simulink model "W06_7_front_vrx"  (R2024b)
settings: Solver=ode4  StartTime=0.0  StopTime=T_run  FixedStep=Ts_ctrl  RelTol=1e-3
InitFcn:
  | if ~exist('W06_model_init','file'), addpath(fileparts(get_param('W06_7_front_vrx','FileName'))); end, W06_model_init('W06_7_front_vrx')
StopFcn:
  | W06_model_done('W06_7_front_vrx')
values from neighbouring files (symbols this model uses):
  alloc_prm = [half_beam; l_bow; F_max; F_bow_max]    [W06_setup.m]
  animate = 0    [W06_bow_demo.m]    (also in W06_psi_sweep.m; W06_setup.m = 1)
  bow_on = BOW(i)    [W06_bow_demo.m]    (also in W06_setup.m = 1)
  F_bow_max = 250    [W06_setup.m]
  F_max = 500    [W06_setup.m]
  F_plugin_max = 2353.53383667818    (= 2353.53383668)    [W06_setup.m]
  half_beam = 1.027135    [W06_setup.m]
  k_prop = 1000 * 0.004422 * 0.2^4    (= 0.0070752)    [W06_setup.m]
  Kb = Ki_u / Kp_u    (= 0.333333333333)    [W06_setup.m]
  Kd_psi = 200    [W06_setup.m]
  Ki_u = 100    [W06_setup.m]
  Ki_v = 100    [W06_setup.m]
  Kp_psi = 400    [W06_setup.m]
  Kp_u = 300    [W06_setup.m]
  Kp_v = 300    [W06_setup.m]
  Kp_x = 0.4    [W06_setup.m]
  Kp_y = 0.4    [W06_setup.m]
  l_bow = 0.75    [W06_setup.m]
  origin_east = -532    [W06_setup.m]
  origin_north = 200    [W06_setup.m]
  stop_hold = 15    [W06_setup.m]
  task_q = [ hold_north;  hold_east;  deg2rad(hold_deg) ... (first row only)    [W06_setup.m]
  Ts_ctrl = 0.05    [W06_setup.m]
  u_max = 1.5    [W06_setup.m]
  v_max = 0.6    [W06_setup.m]
libraries: ros2lib x7, slpidlib x2
settings Model: Creator=admin  LastModifiedBy=admin

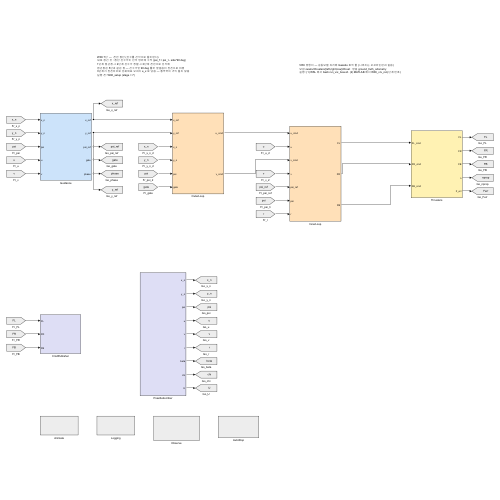
[thumbnail: Simulink's stored preview of the top-level diagram]
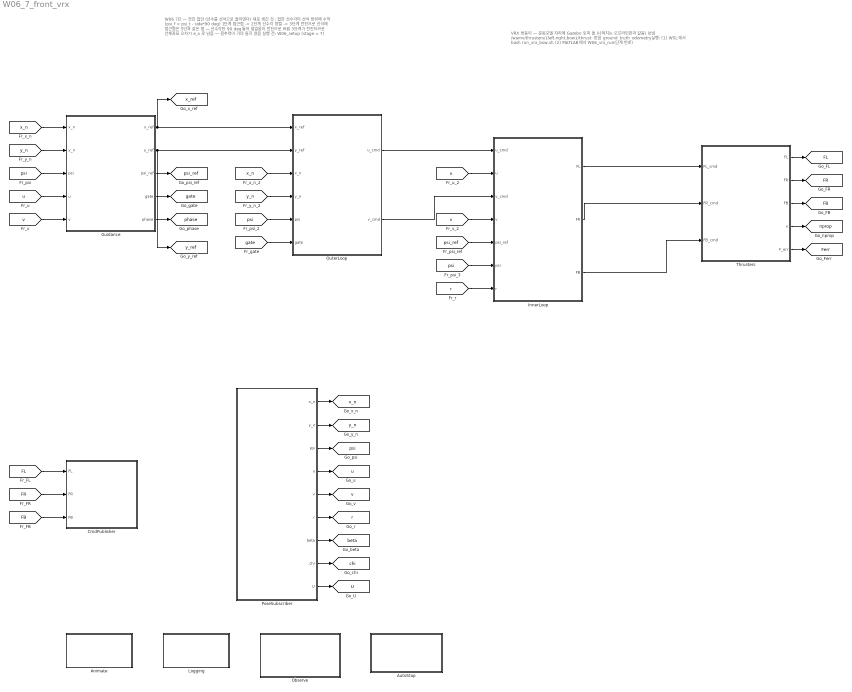
== system W06_7_front_vrx ==
  note: VRX 쌍둥이 — 운동모델 자리에 Gazebo 토픽 둘 (나머지는 오프라인판과 같음)
      | 보냄 /wamv/thrusters/{left,right,bow}/thrust · 받음 ground_truth_odometry
      | 실행: (1) WSL 에서 bash run_vrx_bow.sh  (2) MATLAB 에서 W06_vrx_run(단계 번호)
  note: W06 7단  —  전진 접안 (선수를 선석으로 들이댄다)
      | 새로 생긴 것 : 접안 선수각이 선석 방위에 수직 (psi_f = psi_t - side*90 deg)
      | 1단계 접근점 -> 2단계 선수각 정렬 -> 3단계 전진으로 선석에
      | 접근점은 5단과 같은 점 — 선수각만 90 deg 틀어 옆걸음이 전진으로 바뀜
      | 3단계가 전진이므로 선체좌표 오차가 e_x 로 남음 — 횡추력이 거의 들지 않음
      | 실행 전: W06_setup (stage = 7)
  Animate : Subsystem
  AutoStop : Subsystem
  CmdPublisher : Subsystem
  Guidance : Subsystem
  InnerLoop : Subsystem
  Logging : Subsystem
  Observe : Subsystem
  OuterLoop : Subsystem
  PoseSubscriber : Subsystem
  Thrusters : Subsystem
  tag scope: FB=global, FL=global, FR=global, Ferr=global, U=global, beta=global, chi=global, gate=global, nprop=global, phase=global, psi=global, psi_ref=global, r=global, u=global, v=global, x_n=global, x_ref=global, y_n=global, y_ref=global
  wires:
  InnerLoop/3(FB) -> Thrusters/3(FB_cmd)
  InnerLoop/2(FR) -> Thrusters/2(FR_cmd)
  InnerLoop/1(FL) -> Thrusters/1(FL_cmd)
  OuterLoop/2(v_cmd) -> InnerLoop/3(v_cmd)
  OuterLoop/1(u_cmd) -> InnerLoop/1(u_cmd)
  Guidance/1(x_ref) -> OuterLoop/1(x_ref), [x_ref]
  Guidance/2(y_ref) -> OuterLoop/2(y_ref), [y_ref]
  Thrusters/1(FL) -> [FL]
  Thrusters/2(FR) -> [FR]
  Thrusters/4(n) -> [nprop]
  PoseSubscriber/3(psi) -> [psi]
  Guidance/3(psi_ref) -> [psi_ref]
  PoseSubscriber/6(r) -> [r]
  PoseSubscriber/4(u) -> [u]
  PoseSubscriber/5(v) -> [v]
  PoseSubscriber/1(x_n) -> [x_n]
  PoseSubscriber/2(y_n) -> [y_n]
  [FB] -> CmdPublisher/3(FB)
  [FL] -> CmdPublisher/1(FL)
  [FR] -> CmdPublisher/2(FR)
  [psi_ref] -> InnerLoop/5(psi_ref)
  [r] -> InnerLoop/7(r)
  [u] -> InnerLoop/2(u)
  [v] -> Guidance/5(v)
  [v] -> InnerLoop/4(v)
  [x_n] -> Guidance/1(x_n)
  [y_n] -> Guidance/2(y_n)
  Thrusters/3(FB) -> [FB]
  Thrusters/5(F_err) -> [Ferr]
  PoseSubscriber/9(U) -> [U]
  PoseSubscriber/7(beta) -> [beta]
  PoseSubscriber/8(chi) -> [chi]
  Guidance/4(gate) -> [gate]
  Guidance/5(phase) -> [phase]
  [gate] -> OuterLoop/6(gate)
  [psi] -> Guidance/3(psi)
  [psi] -> InnerLoop/6(psi)
  [u] -> Guidance/4(u)
  [x_n] -> OuterLoop/3(x_n)
  [y_n] -> OuterLoop/4(y_n)
  [psi] -> OuterLoop/5(psi)

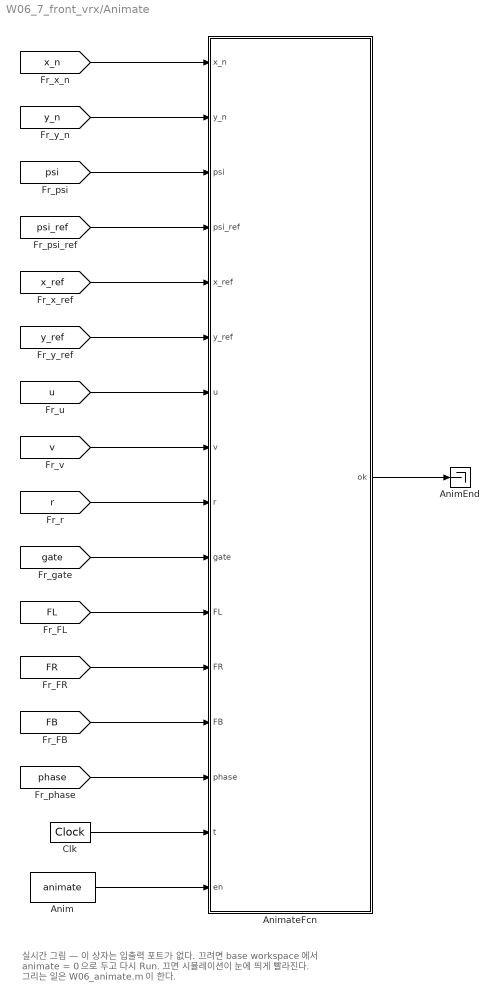
== system W06_7_front_vrx/Animate ==
  note: 실시간 그림 — 이 상자는 입출력 포트가 없다.
      | 끄려면 base workspace 에서  animate = 0  으로 두고 다시 Run.
      | 끄면 시뮬레이션이 눈에 띄게 빨라진다.
      | 그리는 일은 W06_animate.m 이 한다.
  Anim : Constant  Value=animate
  AnimEnd : Terminator
  AnimateFcn : MATLAB Function  TreatAsAtomicUnit=on
  Clk : DigitalClock  SampleTime=Ts_ctrl
  wires:
  [x_n] -> AnimateFcn/1(x_n)
  [y_n] -> AnimateFcn/2(y_n)
  [psi] -> AnimateFcn/3(psi)
  [psi_ref] -> AnimateFcn/4(psi_ref)
  [x_ref] -> AnimateFcn/5(x_ref)
  [y_ref] -> AnimateFcn/6(y_ref)
  [u] -> AnimateFcn/7(u)
  [v] -> AnimateFcn/8(v)
  [r] -> AnimateFcn/9(r)
  [gate] -> AnimateFcn/10(gate)
  [FL] -> AnimateFcn/11(FL)
  [FR] -> AnimateFcn/12(FR)
  [FB] -> AnimateFcn/13(FB)
  [phase] -> AnimateFcn/14(phase)
  Clk/1 -> AnimateFcn/15(t)
  Anim/1 -> AnimateFcn/16(en)
  AnimateFcn/1(ok) -> AnimEnd/1

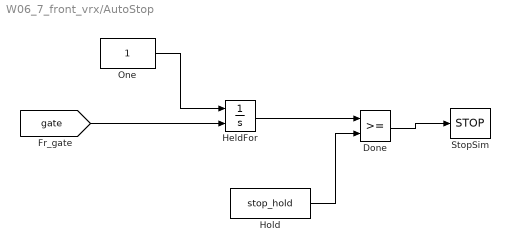
== system W06_7_front_vrx/AutoStop ==
  Done : RelationalOperator  OutDataTypeStr=boolean  RndMeth=Simplest  InputSameDT=off
  HeldFor : Integrator  ExternalReset=level
  Hold : Constant  Value=stop_hold
  One : Constant
  StopSim : Stop
  wires:
  One/1 -> HeldFor/1
  [gate] -> HeldFor/2
  HeldFor/1 -> Done/1
  Hold/1 -> Done/2
  Done/1 -> StopSim/1

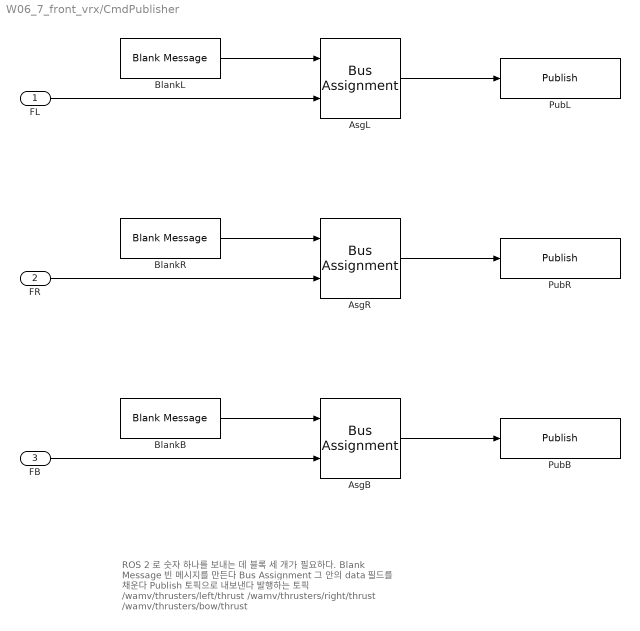
== system W06_7_front_vrx/CmdPublisher ==
  note: ROS 2 로 숫자 하나를 보내는 데 블록 세 개가 필요하다.
      |   Blank Message   빈 메시지를 만든다
      |   Bus Assignment  그 안의 data 필드를 채운다
      |   Publish         토픽으로 내보낸다
      |
      | 발행하는 토픽
      | /wamv/thrusters/left/thrust
      | /wamv/thrusters/right/thrust
      | /wamv/thrusters/bow/thrust
  FL : Inport
  FR : Inport  Port=2
  FB : Inport  Port=3
  AsgB : BusAssignment  AssignedSignals=data
  AsgL : BusAssignment  AssignedSignals=data
  AsgR : BusAssignment  AssignedSignals=data
  BlankB : ros2lib/Blank Message  messageClass=Message  entityType=std_msgs/Float64  messageType=std_msgs/Float64  SampleTime=Ts_ctrl
  BlankL : ros2lib/Blank Message  messageClass=Message  entityType=std_msgs/Float64  messageType=std_msgs/Float64  SampleTime=Ts_ctrl
  BlankR : ros2lib/Blank Message  messageClass=Message  entityType=std_msgs/Float64  messageType=std_msgs/Float64  SampleTime=Ts_ctrl
  PubB : ros2lib/Publish  topicSource=Specify your own  topic=/wamv/thrusters/bow/thrust  messageType=std_msgs/Float64  QOSHistory=Keep last  QOSDepth=1  QOSReliability=Reliable  QOSDurability=Volatile  QOSDeadline=Inf  QOSLifespan=Inf  QOSLiveliness=Automatic  QOSLeaseDuration=Inf  QOSAvoidROSNamespaceConventions=off
  PubL : ros2lib/Publish  topicSource=Specify your own  topic=/wamv/thrusters/left/thrust  messageType=std_msgs/Float64  QOSHistory=Keep last  QOSDepth=1  QOSReliability=Reliable  QOSDurability=Volatile  QOSDeadline=Inf  QOSLifespan=Inf  QOSLiveliness=Automatic  QOSLeaseDuration=Inf  QOSAvoidROSNamespaceConventions=off
  PubR : ros2lib/Publish  topicSource=Specify your own  topic=/wamv/thrusters/right/thrust  messageType=std_msgs/Float64  QOSHistory=Keep last  QOSDepth=1  QOSReliability=Reliable  QOSDurability=Volatile  QOSDeadline=Inf  QOSLifespan=Inf  QOSLiveliness=Automatic  QOSLeaseDuration=Inf  QOSAvoidROSNamespaceConventions=off
  wires:
  BlankL/1 -> AsgL/1
  AsgL/1 -> PubL/1
  FL/1 -> AsgL/2
  BlankR/1 -> AsgR/1
  AsgR/1 -> PubR/1
  FR/1 -> AsgR/2
  BlankB/1 -> AsgB/1
  AsgB/1 -> PubB/1
  FB/1 -> AsgB/2

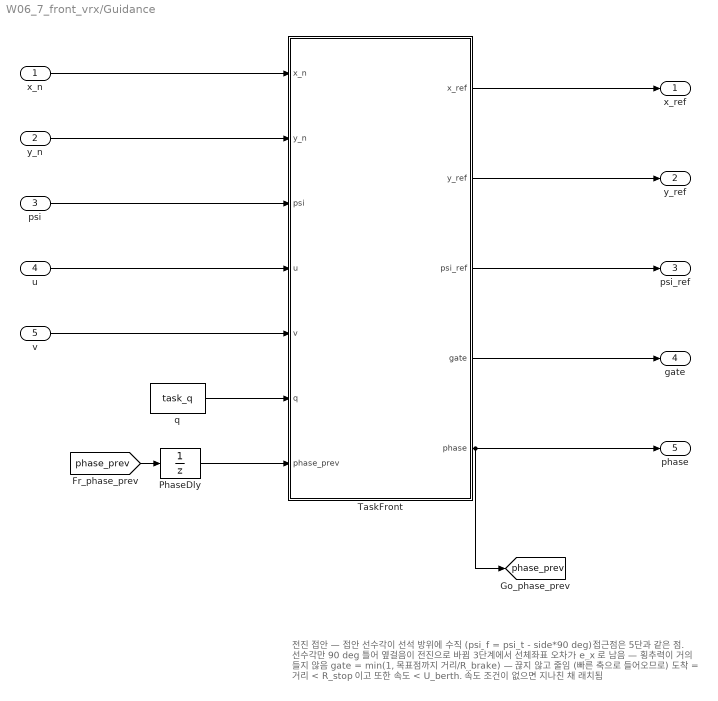
== system W06_7_front_vrx/Guidance ==
  note: 전진 접안 — 접안 선수각이 선석 방위에 수직 (psi_f = psi_t - side*90 deg)
      | 접근점은 5단과 같은 점. 선수각만 90 deg 틀어 옆걸음이 전진으로 바뀜
      | 3단계에서 선체좌표 오차가 e_x 로 남음 — 횡추력이 거의 들지 않음
      | gate = min(1, 목표점까지 거리/R_brake) — 끊지 않고 줄임 (빠른 축으로 들어오므로)
      | 도착 = 거리 < R_stop 이고 또한 속도 < U_berth. 속도 조건이 없으면 지나친 채 래치됨
  x_n : Inport
  y_n : Inport  Port=2
  psi : Inport  Port=3
  u : Inport  Port=4
  v : Inport  Port=5
  PhaseDly : UnitDelay  Description=phase 래치가 자기 자신을 입력으로 받으므로 그대로 되먹이면 대수 루프가 된다. 한 스텝 전 값을 쓰는 것 말고는 끊을 방법이 없는 자리다. 표본 간격을 고정 스텝(Ts_ctrl)과 같게 두어 연속 솔버(ode4)와 어긋나지 않는다.  SampleTime=Ts_ctrl  HasFrameUpgradeWarning=on
  TaskFront : MATLAB Function  TreatAsAtomicUnit=on
  q : Constant  Value=task_q
  x_ref : Outport
  y_ref : Outport  Port=2
  psi_ref : Outport  Port=3
  gate : Outport  Port=4
  phase : Outport  Port=5
  tag scope: phase_prev=global
  wires:
  x_n/1 -> TaskFront/1(x_n)
  y_n/1 -> TaskFront/2(y_n)
  psi/1 -> TaskFront/3(psi)
  u/1 -> TaskFront/4(u)
  v/1 -> TaskFront/5(v)
  q/1 -> TaskFront/6(q)
  PhaseDly/1 -> TaskFront/7(phase_prev)
  TaskFront/1(x_ref) -> x_ref/1
  TaskFront/2(y_ref) -> y_ref/1
  TaskFront/3(psi_ref) -> psi_ref/1
  TaskFront/4(gate) -> gate/1
  TaskFront/5(phase) -> phase/1, [phase_prev]
  [phase_prev] -> PhaseDly/1

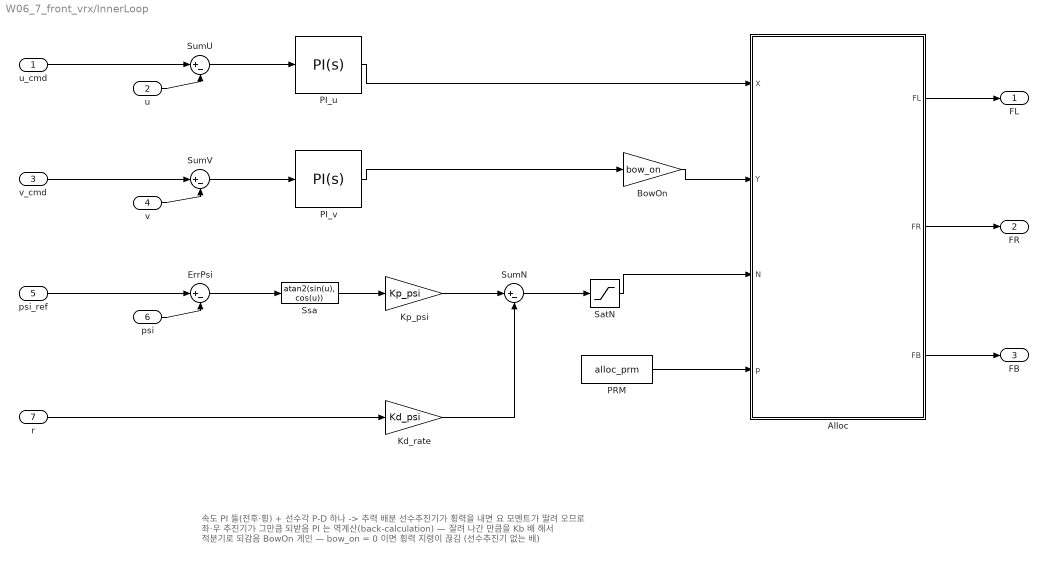
== system W06_7_front_vrx/InnerLoop ==
  note: 속도 PI 둘(전후·횡) + 선수각 P-D 하나 -> 추력 배분
      | 선수추진기가 횡력을 내면 요 모멘트가 딸려 오므로 좌·우 추진기가 그만큼 되받음
      | PI 는 역계산(back-calculation) — 잘려 나간 만큼을 Kb 배 해서 적분기로 되감음
      | BowOn 게인 — bow_on = 0 이면 횡력 지령이 끊김 (선수추진기 없는 배)
  u_cmd : Inport
  u : Inport  Port=2
  v_cmd : Inport  Port=3
  v : Inport  Port=4
  psi_ref : Inport  Port=5
  psi : Inport  Port=6
  r : Inport  Port=7
  Alloc : MATLAB Function  TreatAsAtomicUnit=on
  BowOn : Gain  Gain=bow_on
  ErrPsi : Sum  Inputs=|+-
  Kd_rate : Gain  Gain=Kd_psi
  Kp_psi : Gain  Gain=Kp_psi
  PI_u : slpidlib/PID Controller  Controller=PI  Form=Parallel  TimeDomain=Continuous-time  UseExternalTs=off  SampleTime=-1  IntegratorMethod=Forward Euler  FilterMethod=Forward Euler  ControllerParametersSource=internal  P=Kp_u  I=Ki_u  UseKiTs=off  D=0  UseExternalDerivativeSource=off  N=100  UseFilter=on  TunerSelectOption=Transfer Function Based (PID Tuner App)  InitialConditionSource=internal  InitialConditionForIntegrator=0  InitialConditionForFilter=0  DifferentiatorICPrevScaledInput=0  ExternalReset=none  TrackingMode=off  Kt=1  LimitOutput=on  SatLimitsSource=internal  UpperSaturationLimit=2*F_max  LowerSaturationLimit=-(2*F_max)  LinearizeAsGain=on  AntiWindupMode=back-calculation  Kb=Kb  LimitIntegrator=off  UpperIntegratorSaturationLimit=inf  LowerIntegratorSaturationLimit=-inf  POutMin=[]  POutMax=[]  IOutMin=[]  IOutMax=[]  DOutMin=[]  DOutMax=[]  NOutMin=[]  NOutMax=[]  SumOutMin=[]  SumOutMax=[]  SaturationOutMin=[]  SaturationOutMax=[]  PParamMin=[]  PParamMax=[]  IParamMin=[]  IParamMax=[]  DParamMin=[]  DParamMax=[]  NParamMin=[]  NParamMax=[]  KbParamMin=[]  KbParamMax=[]  KtParamMin=[]  KtParamMax=[]  KbOutMin=[]  KbOutMax=[]  KtOutMin=[]  KtOutMax=[]  IntegratorOutMin=[]  IntegratorOutMax=[]  FilterOutMin=[]  FilterOutMax=[]  SumI1OutMin=[]  SumI1OutMax=[]  SumI2OutMin=[]  SumI2OutMax=[]  SumI3OutMin=[]  SumI3OutMax=[]  SumI4OutMin=[]  SumI4OutMax=[]  SumDOutMin=[]  SumDOutMax=[]  DifferentiatorOutMin=[]  DifferentiatorOutMax=[]  FilterDiffOutCoefMin=[]  FilterDiffOutCoefMax=[]  ReciprocalOutMin=[]  ReciprocalOutMax=[]  SumDenOutMin=[]  SumDenOutMax=[]  SumNumOutMin=[]  SumNumOutMax=[]  DivideOutMin=[]  DivideOutMax=[]  UdiffTsProdOutMin=[]  UdiffTsProdOutMax=[]  NTsProdOutMin=[]  NTsProdOutMax=[]  UintegralTsProdOutMin=[]  UintegralTsProdOutMax=[]  UngainTsProdOutMin=[]  UngainTsProdOutMax=[]  ClampingZeroOutDataTypeStr=Inherit: Inherit via back propagation  ClampingZeroOutMin=[]  ClampingZeroOutMax=[]  FilterDenConstantOutDataTypeStr=Inherit: Inherit via back propagation  FilterDenConstantOutMin=[]  FilterDenConstantOutMax=[]  PCopyOutDataTypeStr=Inherit: Inherit via back propagation  PCopyOutMin=[]  PCopyOutMax=[]  NCopyOutDataTypeStr=Inherit: Inherit via back propagation  NCopyOutMin=[]  NCopyOutMax=[]  IntegratorContinuousStateAttributes=''  IntegratorStateMustResolveToSignalObject=off  IntegratorRTWStateStorageClass=Auto  FilterContinuousStateAttributes=''  FilterStateMustResolveToSignalObject=off  FilterRTWStateStorageClass=Auto  ParallelPVariant=InternalParameters  IdealPVariant=Disabled  IVariant=InternalParameters  DVariant=Disabled  IntegratorVariant=Continuous  SatVariant=Enabled  AWVariant=BackCalculation  PCopyVariant=Disabled  TRVariant=Disabled  FdbkBlocksVariant=Forward  IdealPFdbkVariant=Disabled  SatFdbkVariant=Disabled  DerivativeFilterVariant=Disabled  NVariant=Disabled  NCopyVariant=Disabled_SignalSpec  FilterICVariant=Disabled  IntegratorICVariant=InternalICs  ExternalResetVariant=Disabled  TRSumVariant=Passthrough  SumFdbkVariant=Disabled  SumVariant=Sum_PI  TsampFilterVariant=InternalTs  TsampNgainVariant=Passthrough  TsampIntegralVariant=Disabled_SignalSpec  ExternalSaturationOutDataTypeStr=Inherit: Same as second input  DerivativeSourceVariant=Disabled  PreIntVariant=InternalPreInt
  PI_v : slpidlib/PID Controller  Controller=PI  Form=Parallel  TimeDomain=Continuous-time  UseExternalTs=off  SampleTime=-1  IntegratorMethod=Forward Euler  FilterMethod=Forward Euler  ControllerParametersSource=internal  P=Kp_v  I=Ki_v  UseKiTs=off  D=0  UseExternalDerivativeSource=off  N=100  UseFilter=on  TunerSelectOption=Transfer Function Based (PID Tuner App)  InitialConditionSource=internal  InitialConditionForIntegrator=0  InitialConditionForFilter=0  DifferentiatorICPrevScaledInput=0  ExternalReset=none  TrackingMode=off  Kt=1  LimitOutput=on  SatLimitsSource=internal  UpperSaturationLimit=F_bow_max  LowerSaturationLimit=-(F_bow_max)  LinearizeAsGain=on  AntiWindupMode=back-calculation  Kb=Kb  LimitIntegrator=off  UpperIntegratorSaturationLimit=inf  LowerIntegratorSaturationLimit=-inf  POutMin=[]  POutMax=[]  IOutMin=[]  IOutMax=[]  DOutMin=[]  DOutMax=[]  NOutMin=[]  NOutMax=[]  SumOutMin=[]  SumOutMax=[]  SaturationOutMin=[]  SaturationOutMax=[]  PParamMin=[]  PParamMax=[]  IParamMin=[]  IParamMax=[]  DParamMin=[]  DParamMax=[]  NParamMin=[]  NParamMax=[]  KbParamMin=[]  KbParamMax=[]  KtParamMin=[]  KtParamMax=[]  KbOutMin=[]  KbOutMax=[]  KtOutMin=[]  KtOutMax=[]  IntegratorOutMin=[]  IntegratorOutMax=[]  FilterOutMin=[]  FilterOutMax=[]  SumI1OutMin=[]  SumI1OutMax=[]  SumI2OutMin=[]  SumI2OutMax=[]  SumI3OutMin=[]  SumI3OutMax=[]  SumI4OutMin=[]  SumI4OutMax=[]  SumDOutMin=[]  SumDOutMax=[]  DifferentiatorOutMin=[]  DifferentiatorOutMax=[]  FilterDiffOutCoefMin=[]  FilterDiffOutCoefMax=[]  ReciprocalOutMin=[]  ReciprocalOutMax=[]  SumDenOutMin=[]  SumDenOutMax=[]  SumNumOutMin=[]  SumNumOutMax=[]  DivideOutMin=[]  DivideOutMax=[]  UdiffTsProdOutMin=[]  UdiffTsProdOutMax=[]  NTsProdOutMin=[]  NTsProdOutMax=[]  UintegralTsProdOutMin=[]  UintegralTsProdOutMax=[]  UngainTsProdOutMin=[]  UngainTsProdOutMax=[]  ClampingZeroOutDataTypeStr=Inherit: Inherit via back propagation  ClampingZeroOutMin=[]  ClampingZeroOutMax=[]  FilterDenConstantOutDataTypeStr=Inherit: Inherit via back propagation  FilterDenConstantOutMin=[]  FilterDenConstantOutMax=[]  PCopyOutDataTypeStr=Inherit: Inherit via back propagation  PCopyOutMin=[]  PCopyOutMax=[]  NCopyOutDataTypeStr=Inherit: Inherit via back propagation  NCopyOutMin=[]  NCopyOutMax=[]  IntegratorContinuousStateAttributes=''  IntegratorStateMustResolveToSignalObject=off  IntegratorRTWStateStorageClass=Auto  FilterContinuousStateAttributes=''  FilterStateMustResolveToSignalObject=off  FilterRTWStateStorageClass=Auto  ParallelPVariant=InternalParameters  IdealPVariant=Disabled  IVariant=InternalParameters  DVariant=Disabled  IntegratorVariant=Continuous  SatVariant=Enabled  AWVariant=BackCalculation  PCopyVariant=Disabled  TRVariant=Disabled  FdbkBlocksVariant=Forward  IdealPFdbkVariant=Disabled  SatFdbkVariant=Disabled  DerivativeFilterVariant=Disabled  NVariant=Disabled  NCopyVariant=Disabled_SignalSpec  FilterICVariant=Disabled  IntegratorICVariant=InternalICs  ExternalResetVariant=Disabled  TRSumVariant=Passthrough  SumFdbkVariant=Disabled  SumVariant=Sum_PI  TsampFilterVariant=InternalTs  TsampNgainVariant=Passthrough  TsampIntegralVariant=Disabled_SignalSpec  ExternalSaturationOutDataTypeStr=Inherit: Same as second input  DerivativeSourceVariant=Disabled  PreIntVariant=InternalPreInt
  PRM : Constant  Value=alloc_prm
  SatN : Saturate  UpperLimit=2*F_max*half_beam + F_bow_max*l_bow  LowerLimit=-(2*F_max*half_beam + F_bow_max*l_bow)
  Ssa : Fcn  Expr=atan2(sin(u), cos(u))
  SumN : Sum  Inputs=|+-
  SumU : Sum  Inputs=|+-
  SumV : Sum  Inputs=|+-
  FL : Outport
  FR : Outport  Port=2
  FB : Outport  Port=3
  wires:
  u_cmd/1 -> SumU/1
  u/1 -> SumU/2
  v_cmd/1 -> SumV/1
  v/1 -> SumV/2
  SumU/1 -> PI_u/1
  SumV/1 -> PI_v/1
  ErrPsi/1 -> Ssa/1
  psi_ref/1 -> ErrPsi/1
  psi/1 -> ErrPsi/2
  Ssa/1 -> Kp_psi/1
  r/1 -> Kd_rate/1
  Kp_psi/1 -> SumN/1
  Kd_rate/1 -> SumN/2
  SumN/1 -> SatN/1
  PI_u/1 -> Alloc/1(X)
  PI_v/1 -> BowOn/1
  BowOn/1 -> Alloc/2(Y)
  SatN/1 -> Alloc/3(N)
  PRM/1 -> Alloc/4(p)
  Alloc/1(FL) -> FL/1
  Alloc/2(FR) -> FR/1
  Alloc/3(FB) -> FB/1

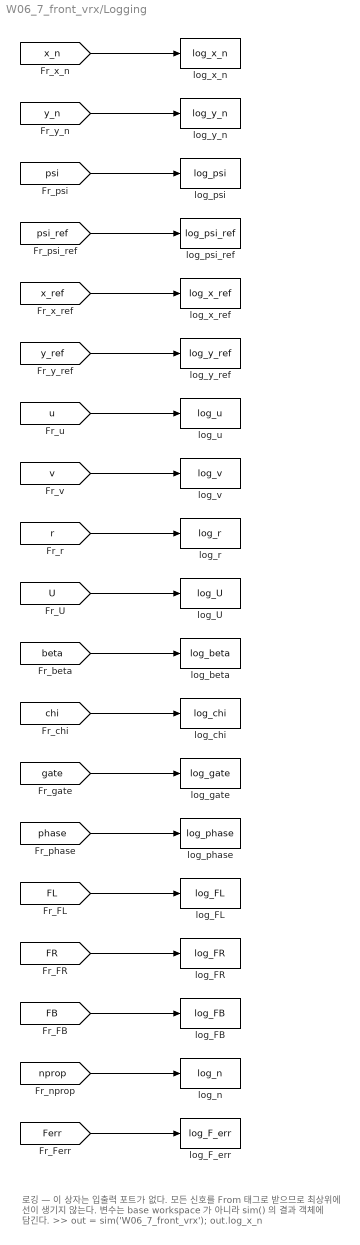
== system W06_7_front_vrx/Logging ==
  note: 로깅 — 이 상자는 입출력 포트가 없다.
      | 모든 신호를 From 태그로 받으므로 최상위에 선이 생기지 않는다.
      | 변수는 base workspace 가 아니라 sim() 의 결과 객체에 담긴다.
      |   >> out = sim('W06_7_front_vrx');  out.log_x_n
  log_FB : ToWorkspace  VariableName=log_FB  SaveFormat=Timeseries  SampleTime=Ts_ctrl
  log_FL : ToWorkspace  VariableName=log_FL  SaveFormat=Timeseries  SampleTime=Ts_ctrl
  log_FR : ToWorkspace  VariableName=log_FR  SaveFormat=Timeseries  SampleTime=Ts_ctrl
  log_F_err : ToWorkspace  VariableName=log_F_err  SaveFormat=Timeseries  SampleTime=Ts_ctrl
  log_U : ToWorkspace  VariableName=log_U  SaveFormat=Timeseries  SampleTime=Ts_ctrl
  log_beta : ToWorkspace  VariableName=log_beta  SaveFormat=Timeseries  SampleTime=Ts_ctrl
  log_chi : ToWorkspace  VariableName=log_chi  SaveFormat=Timeseries  SampleTime=Ts_ctrl
  log_gate : ToWorkspace  VariableName=log_gate  SaveFormat=Timeseries  SampleTime=Ts_ctrl
  log_n : ToWorkspace  VariableName=log_n  SaveFormat=Timeseries  SampleTime=Ts_ctrl
  log_phase : ToWorkspace  VariableName=log_phase  SaveFormat=Timeseries  SampleTime=Ts_ctrl
  log_psi : ToWorkspace  VariableName=log_psi  SaveFormat=Timeseries  SampleTime=Ts_ctrl
  log_psi_ref : ToWorkspace  VariableName=log_psi_ref  SaveFormat=Timeseries  SampleTime=Ts_ctrl
  log_r : ToWorkspace  VariableName=log_r  SaveFormat=Timeseries  SampleTime=Ts_ctrl
  log_u : ToWorkspace  VariableName=log_u  SaveFormat=Timeseries  SampleTime=Ts_ctrl
  log_v : ToWorkspace  VariableName=log_v  SaveFormat=Timeseries  SampleTime=Ts_ctrl
  log_x_n : ToWorkspace  VariableName=log_x_n  SaveFormat=Timeseries  SampleTime=Ts_ctrl
  log_x_ref : ToWorkspace  VariableName=log_x_ref  SaveFormat=Timeseries  SampleTime=Ts_ctrl
  log_y_n : ToWorkspace  VariableName=log_y_n  SaveFormat=Timeseries  SampleTime=Ts_ctrl
  log_y_ref : ToWorkspace  VariableName=log_y_ref  SaveFormat=Timeseries  SampleTime=Ts_ctrl
  wires:
  [x_n] -> log_x_n/1
  [y_n] -> log_y_n/1
  [psi] -> log_psi/1
  [psi_ref] -> log_psi_ref/1
  [x_ref] -> log_x_ref/1
  [y_ref] -> log_y_ref/1
  [u] -> log_u/1
  [v] -> log_v/1
  [r] -> log_r/1
  [U] -> log_U/1
  [beta] -> log_beta/1
  [chi] -> log_chi/1
  [gate] -> log_gate/1
  [phase] -> log_phase/1
  [FL] -> log_FL/1
  [FR] -> log_FR/1
  [FB] -> log_FB/1
  [nprop] -> log_n/1
  [Ferr] -> log_F_err/1

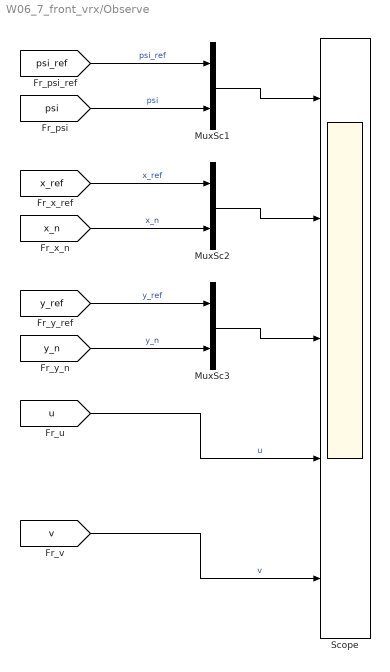
== system W06_7_front_vrx/Observe ==
  MuxSc1 : Mux  Inputs=2
  MuxSc2 : Mux  Inputs=2
  MuxSc3 : Mux  Inputs=2
  Scope : Scope  NumInputPorts=5
  wires:
  [psi_ref] -> MuxSc1/1  "psi_ref"
  [psi] -> MuxSc1/2  "psi"
  MuxSc1/1 -> Scope/1
  [x_ref] -> MuxSc2/1  "x_ref"
  [x_n] -> MuxSc2/2  "x_n"
  MuxSc2/1 -> Scope/2
  [y_ref] -> MuxSc3/1  "y_ref"
  [y_n] -> MuxSc3/2  "y_n"
  MuxSc3/1 -> Scope/3
  [u] -> Scope/4  "u"
  [v] -> Scope/5  "v"

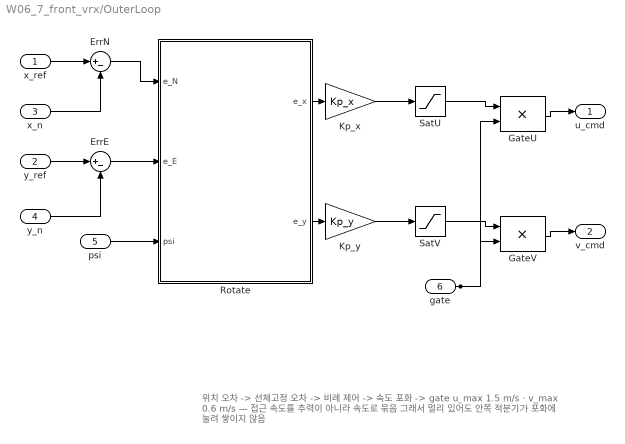
== system W06_7_front_vrx/OuterLoop ==
  note: 위치 오차 -> 선체고정 오차 -> 비례 제어 -> 속도 포화 -> gate
      | u_max 1.5 m/s · v_max 0.6 m/s — 접근 속도를 추력이 아니라 속도로 묶음
      | 그래서 멀리 있어도 안쪽 적분기가 포화에 눌려 쌓이지 않음
  x_ref : Inport
  y_ref : Inport  Port=2
  x_n : Inport  Port=3
  y_n : Inport  Port=4
  psi : Inport  Port=5
  gate : Inport  Port=6
  ErrE : Sum  Inputs=|+-
  ErrN : Sum  Inputs=|+-
  GateU : Product
  GateV : Product
  Kp_x : Gain  Gain=Kp_x
  Kp_y : Gain  Gain=Kp_y
  Rotate : MATLAB Function  TreatAsAtomicUnit=on
  SatU : Saturate  UpperLimit=u_max  LowerLimit=-(u_max)
  SatV : Saturate  UpperLimit=v_max  LowerLimit=-(v_max)
  u_cmd : Outport
  v_cmd : Outport  Port=2
  wires:
  psi/1 -> Rotate/3(psi)
  Rotate/1(e_x) -> Kp_x/1
  GateU/1 -> u_cmd/1
  x_ref/1 -> ErrN/1
  x_n/1 -> ErrN/2
  y_ref/1 -> ErrE/1
  y_n/1 -> ErrE/2
  ErrN/1 -> Rotate/1(e_N)
  ErrE/1 -> Rotate/2(e_E)
  Rotate/2(e_y) -> Kp_y/1
  SatV/1 -> GateV/1
  Kp_x/1 -> SatU/1
  Kp_y/1 -> SatV/1
  SatU/1 -> GateU/1
  gate/1 -> GateU/2, GateV/2
  GateV/1 -> v_cmd/1

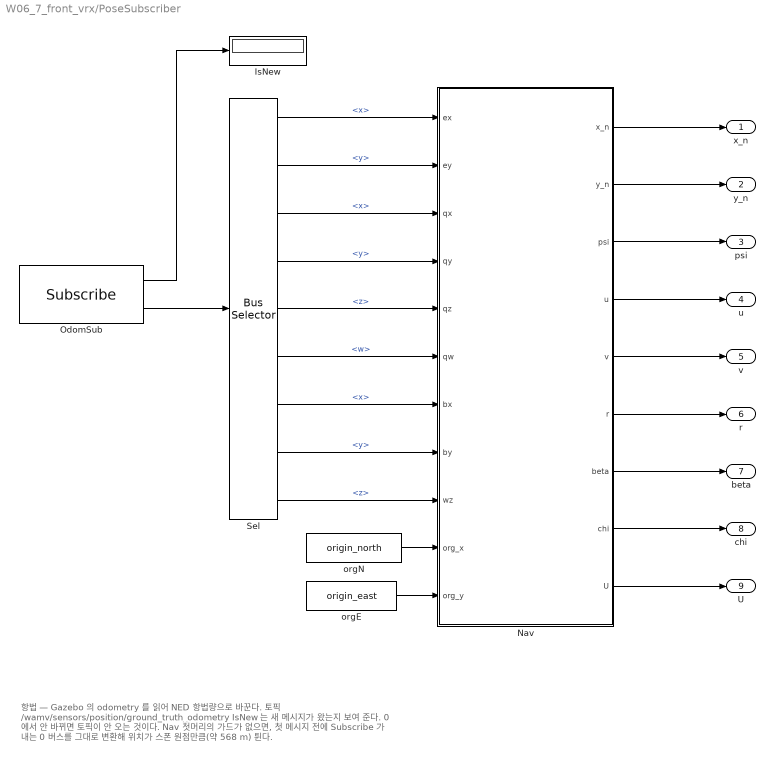
== system W06_7_front_vrx/PoseSubscriber ==
  note: 항법 — Gazebo 의 odometry 를 읽어 NED 항법량으로 바꾼다.
      |   토픽 /wamv/sensors/position/ground_truth_odometry
      |
      | IsNew 는 새 메시지가 왔는지 보여 준다. 0 에서 안 바뀌면 토픽이 안 오는 것이다.
      | Nav 첫머리의 가드가 없으면, 첫 메시지 전에 Subscribe 가 내는 0 버스를
      | 그대로 변환해 위치가 스폰 원점만큼(약 568 m) 튄다.
  IsNew : Display
  Nav : MATLAB Function  TreatAsAtomicUnit=on
  OdomSub : ros2lib/Subscribe  topicSource=Specify your own  topic=/wamv/sensors/position/ground_truth_odometry  messageType=nav_msgs/Odometry  sampleTime=Ts_ctrl  QOSHistory=Keep last  QOSDepth=1  QOSReliability=Reliable  QOSDurability=Volatile  QOSDeadline=Inf  QOSLifespan=Inf  QOSLiveliness=Automatic  QOSLeaseDuration=Inf  QOSAvoidROSNamespaceConventions=off
  Sel : BusSelector  OutputSignals=pose.pose.position.x,pose.pose.position.y,pose.pose.orientation.x,pose.pose.orientation.y,pose.pose.orientation.z,pose.pose.orientation.w,twist.twist.linear.x,twist.twist.linear.y,twist.twist.angular.z
  orgE : Constant  Value=origin_east
  orgN : Constant  Value=origin_north
  x_n : Outport
  y_n : Outport  Port=2
  psi : Outport  Port=3
  u : Outport  Port=4
  v : Outport  Port=5
  r : Outport  Port=6
  beta : Outport  Port=7
  chi : Outport  Port=8
  U : Outport  Port=9
  wires:
  OdomSub/1 -> IsNew/1
  OdomSub/2 -> Sel/1
  Sel/1 -> Nav/1(ex)  "<x>"
  Sel/2 -> Nav/2(ey)  "<y>"
  Sel/3 -> Nav/3(qx)  "<x>"
  Sel/4 -> Nav/4(qy)  "<y>"
  Sel/5 -> Nav/5(qz)  "<z>"
  Sel/6 -> Nav/6(qw)  "<w>"
  Sel/7 -> Nav/7(bx)  "<x>"
  Sel/8 -> Nav/8(by)  "<y>"
  Sel/9 -> Nav/9(wz)  "<z>"
  orgN/1 -> Nav/10(org_x)
  orgE/1 -> Nav/11(org_y)
  Nav/1(x_n) -> x_n/1
  Nav/2(y_n) -> y_n/1
  Nav/3(psi) -> psi/1
  Nav/4(u) -> u/1
  Nav/5(v) -> v/1
  Nav/6(r) -> r/1
  Nav/7(beta) -> beta/1
  Nav/8(chi) -> chi/1
  Nav/9(U) -> U/1

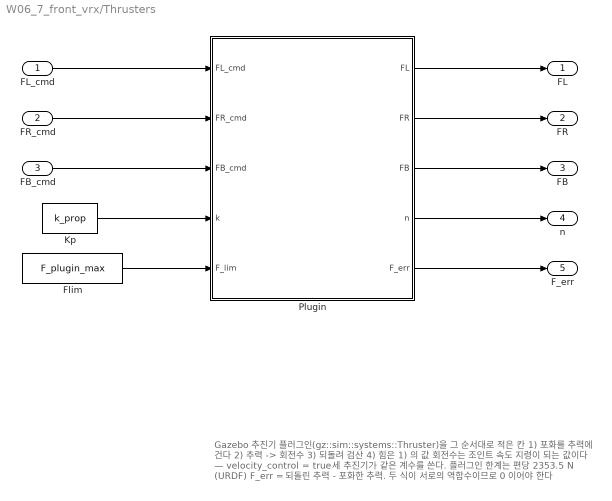
== system W06_7_front_vrx/Thrusters ==
  note: Gazebo 추진기 플러그인(gz::sim::systems::Thruster)을 그 순서대로 적은 칸
      | 1) 포화를 추력에 건다  2) 추력 -> 회전수  3) 되돌려 검산  4) 힘은 1) 의 값
      | 회전수는 조인트 속도 지령이 되는 값이다 — velocity_control = true
      | 세 추진기가 같은 계수를 쓴다. 플러그인 한계는 편당 2353.5 N (URDF)
      | F_err = 되돌린 추력 - 포화한 추력. 두 식이 서로의 역함수이므로 0 이어야 한다
  FL_cmd : Inport
  FR_cmd : Inport  Port=2
  FB_cmd : Inport  Port=3
  Flim : Constant  Value=F_plugin_max
  Kp : Constant  Value=k_prop
  Plugin : MATLAB Function  TreatAsAtomicUnit=on
  FL : Outport
  FR : Outport  Port=2
  FB : Outport  Port=3
  n : Outport  Port=4
  F_err : Outport  Port=5
  wires:
  FL_cmd/1 -> Plugin/1(FL_cmd)
  FR_cmd/1 -> Plugin/2(FR_cmd)
  FB_cmd/1 -> Plugin/3(FB_cmd)
  Kp/1 -> Plugin/4(k)
  Flim/1 -> Plugin/5(F_lim)
  Plugin/1(FL) -> FL/1
  Plugin/2(FR) -> FR/1
  Plugin/3(FB) -> FB/1
  Plugin/4(n) -> n/1
  Plugin/5(F_err) -> F_err/1

== matlab function W06_7_front_vrx/Animate/AnimateFcn ==
  data: x_n input; y_n input; psi input; psi_ref input; x_ref input; y_ref input; u input; ok output; v input; r input; gate input; FL input; FR input; FB input; phase input; t input; en input
function ok = AnimateFcn(x_n, y_n, psi, psi_ref, x_ref, y_ref, u, v, r, gate, FL, FR, FB, phase, t, en)
%#codegen
% Live plot while the model runs. A MATLAB Function block cannot
% plot, so the drawing function is declared extrinsic: Simulink
% calls plain MATLAB instead of generating code for it.
coder.extrinsic('W06_animate');
ok = 1;
if en > 0.5
    W06_animate(x_n, y_n, psi, psi_ref, x_ref, y_ref, u, v, r, gate, FL, FR, FB, phase, t);
end

== matlab function W06_7_front_vrx/OuterLoop/Rotate ==
  data: e_N input; e_x output; e_E input; psi input; e_y output
function [e_x, e_y] = Rotate(e_N, e_E, psi)
%#codegen
%  NED 위치 오차를 선체고정 오차로 돌린다. e_x 앞쪽, e_y 우현쪽 [m]
e_x =  cos(psi)*e_N + sin(psi)*e_E;
e_y = -sin(psi)*e_N + cos(psi)*e_E;

== matlab function W06_7_front_vrx/Guidance/TaskFront ==
  data: x_n input; y_n input; psi input; u input; x_ref output; v input; q input; phase_prev input; y_ref output; psi_ref output; gate output; phase output
function [x_ref, y_ref, psi_ref, gate, phase] = TaskFront(x_n, y_n, psi, u, v, q, phase_prev)
%#codegen
%  전진 접안(bow-first)이 요구하는 목표 자세와 진행 단계를 내놓는다.
%
%    q(7:9)   접안 목표       north, east, 선석 방위 [rad]
%    q(10)    R_dock      접근점에 닿았다고 보는 반지름 [m]
%    q(11)    L_app       접안점에서 접근점까지의 거리 [m]
%    q(12)    berth_side  +1 이면 부두가 좌현쪽
%    q(13)    R_stop      접안점에 닿았다고 보는 반지름 [m]
%    q(15)    R_brake     이 거리 안에서 접근 속도를 줄인다 [m]
%    q(16)    U_berth     도착으로 보는 속도 한계 [m/s]
%
%  gate 는 0/1 스위치가 아니라 감속 계수다 — 목표점까지 거리에 비례해
%  속도 지령을 줄이고, 도착(가깝고 느림)하면 0 으로 래치한다.
dx = q(7);  dy = q(8);  dpsi = q(9);
Rd = q(10); La = q(11); sd = q(12); Rs = q(13);
Rb = q(15); Ub = q(16);

%  접안 선수각 — 선석 방위에 수직. 선수가 부두를 향한다
psi_f = dpsi - sd*pi/2;

%  접근점 — 접안점에서 접안 선수각의 뒤쪽으로 L_app (논문 식 5)
ax = dx - La*cos(psi_f);
ay = dy - La*sin(psi_f);

ph = phase_prev;
if ph < 1
    %  1단계 — 접근점으로 간다. 선수각은 가는 방향으로 둔다 (저항이 작다)
    x_ref = ax;  y_ref = ay;
    psi_ref = atan2(ay - y_n, ax - x_n);
    if sqrt((ax - x_n)^2 + (ay - y_n)^2) < Rd
        ph = 1;
    end
elseif ph < 2
    %  2단계 — 접근점에 머물며 선수각만 접안 선수각으로 돌린다
    x_ref = ax;  y_ref = ay;  psi_ref = psi_f;
    e = atan2(sin(psi_f - psi), cos(psi_f - psi));
    if abs(e) < 5*pi/180
        ph = 2;
    end
else
    %  3단계 — 선수각을 지킨 채 전진으로 접안점에 붙인다
    x_ref = dx;  y_ref = dy;  psi_ref = psi_f;
    %  도착 = 가깝고 **거의 멈춰** 있을 때. 속도 조건이 없으면 빠르게
    %  지나가는 순간에 래치되어 지나친 오차를 되돌릴 길이 없어진다
    if sqrt((dx - x_n)^2 + (dy - y_n)^2) < Rs && sqrt(u^2 + v^2) < Ub
        ph = 3;
    end
end
phase = ph;

%  감속 — 목표점까지 거리가 R_brake 안으로 들면 속도 지령을 깎는다.
%  바깥 고리의 비례 제어와 겹쳐 지령이 거리의 제곱으로 떨어지므로,
%  지령이 실제 속도보다 먼저 내려가 속도 PI 의 적분이 되감긴다.
if ph < 3
    d_t = sqrt((x_ref - x_n)^2 + (y_ref - y_n)^2);
    gate = min(1, d_t / Rb);
else
    gate = 0;
end

== matlab function W06_7_front_vrx/InnerLoop/Alloc ==
  data: X input; FL output; Y input; N input; p input; FR output; FB output
function [FL, FR, FB] = Alloc(X, Y, N, p)
%#codegen
%  추력 배분 — 요구 힘·모멘트를 세 추진기로 나눈다.
%
%    X = FL + FR                      전후력 [N]
%    Y = FB                           횡력 [N]  — 선수추진기만 낸다
%    N = (FL - FR)*b + l3*FB          요 모멘트 [N m]
%
%  p = [b; l3; Fmax; Fbmax]
%    b     half_beam   좌·우 추진기까지의 반폭 [m]
%    l3    l_bow       무게중심에서 선수추진기까지 [m]
%    Fmax  선미 추진기 추력 한계 [N],  Fbmax 선수추진기 추력 한계 [N]
%
%  선수추진기가 횡력을 내면 요 모멘트 l3*FB 가 딸려 온다. 그것을 좌·우
%  추진기가 되받아 빼야 선수각이 돌아가지 않는다 — 아래 N - l3*FB 가 그것이다.
b = p(1);  l3 = p(2);  Fmax = p(3);  Fbmax = p(4);
FB = Y;
if FB >  Fbmax, FB =  Fbmax; end
if FB < -Fbmax, FB = -Fbmax; end
%  포화된 뒤의 FB 로 모멘트를 센다 — 실제로 딸려 온 만큼만 되받는다
M  = N - l3*FB;
FL = X/2 + M/(2*b);
FR = X/2 - M/(2*b);
if FL >  Fmax, FL =  Fmax; end
if FL < -Fmax, FL = -Fmax; end
if FR >  Fmax, FR =  Fmax; end
if FR < -Fmax, FR = -Fmax; end

== matlab function W06_7_front_vrx/Thrusters/Plugin ==
  data: FL_cmd input; FL output; FR_cmd input; FB_cmd input; k input; F_lim input; FR output; FB output; n output; F_err output
function [FL, FR, FB, n, F_err] = Plugin(FL_cmd, FR_cmd, FB_cmd, k, F_lim)
%#codegen
%  Gazebo 추진기 플러그인이 하는 일을 소스와 같은 순서로 적는다.
%    gz-sim7  src/systems/thruster/Thruster.cc

%  1) 포화 — 플러그인은 **추력에** 건다 (OnCmdThrust, :520-521)
%       thrust = clamp(cmd, cmdMin, cmdMax),  cmdMax = max_thrust_cmd
F = [FL_cmd; FR_cmd; FB_cmd];
F = max(-F_lim, min(F_lim, F));

%  2) 추력 -> 회전수 (ThrustToAngularVec, :562-584). 이 값이 조인트
%     속도 지령이 된다 — velocity_control = true (:740-756)
%       omega = sign(F*Ct)*sqrt(|F|/(rho*Ct*D^4)),  k = rho*Ct*D^4
%     Ct > 0 이므로 sign(F*Ct) = sign(F) 다
n = sign(F) .* sqrt(abs(F)/k);

%  3) 회전수 -> 추력 (AngularVelToThrust, :593-599). 플러그인에서는
%     회전수 지령 모드에만 쓰인다. 여기서는 2) 를 되돌려 맞는지 보는
%     **검산**이다 — 두 식이 서로의 역함수이므로 0 이 나와야 한다
%       F = rho*Ct*D^4 * |omega| * omega
F_chk = k * abs(n) .* n;
F_err = F_chk - F;

%  4) 링크에 가는 힘은 되돌린 값이 아니라 포화만 거친 지령이다
%     (AddWorldWrench 가 desiredThrust 를 그대로 쓴다, :770-773)
FL = F(1);
FR = F(2);
FB = F(3);

== matlab function W06_7_front_vrx/PoseSubscriber/Nav ==
  data: ex input; x_n output; ey input; qx input; qy input; qz input; qw input; bx input; by input; wz input; org_x input; org_y input; y_n output; psi output; u output; v output; r output; beta output; chi output; U output
function [x_n, y_n, psi, u, v, r, beta, chi, U] = Nav(ex, ey, qx, qy, qz, qw, bx, by, wz, org_x, org_y)
%#codegen
%  Gazebo/ROS 는 ENU 에 선체축 x 앞 · y 좌현 · z 위.
%  해양제어는 NED 에 선체축 x 앞 · y 우현 · z 아래.
%
%    위치   : 북 = y_ENU,  동 = x_ENU   (스폰 원점을 뺀다)
%    선수각 : psi = pi/2 - yaw_ENU
%    선체속도: u = bx,  v = -by,  r = -wz   (y·z 부호가 바뀐다)

%  첫 메시지가 오기 전 Subscribe 는 0 으로 채운 버스를 낸다. 그대로 쓰면
%  위치가 스폰 원점만큼(약 568 m) 튀어 로그 첫 점이 망가진다.
if ex == 0 && ey == 0
    x_n = 0; y_n = 0; psi = 0; u = 0; v = 0; r = 0; beta = 0; chi = 0; U = 0;
    return
end
x_n = ey - org_x;    % north, 스폰 기준 상대좌표
y_n = ex - org_y;    % east

yaw_enu = atan2(2*(qw*qz + qx*qy), 1 - 2*(qy*qy + qz*qz));
p   = pi/2 - yaw_enu;
psi = atan2(sin(p), cos(p));

u = bx;
v = -by;
r = -wz;

U    = sqrt(u*u + v*v);
beta = atan2(v, u);          % 크랩각
c    = psi + beta;
chi  = atan2(sin(c), cos(c));
